simulink model "toa_wl00"  (Simulink 9.0)
settings: Solver=FixedStepDiscrete  StartTime=0.0  StopTime=inf  FixedStep=0.02  RelTol=1e-3  EnableMultiTasking=on
PreLoadFcn:
  | makefile_build_callback(bdroot,'toa_wl00.buildescription');
libraries: lib_CATutils_Utilities_ApplyName_v2 x3, package_instance x1, tip_assist_lib_support x1
settings Model: LogicAnalyzerSignalOrdering=5984164a-15a1-47b0-834b-00decfb9521f  MinMaxOverflowLogging=MinMaxAndOverflow  Creator=gulamhs  LastModifiedBy=CurriSD
settings DataIOCC: ExternalInput=[t,u]  SaveCompleteFinalSimState=on  SaveFormat=StructureWithTime  SaveOutput=off  SignalLogging=off  DSMLogging=off  SaveTime=off
settings OptimizationCC: DefaultParameterBehavior=Inlined  InlineInvariantSignals=on  EnhancedBackFolding=on  StrengthReduction=on  BitfieldContainerType=uchar_T  PassReuseOutputArgsAs=Individual arguments  ExpressionDepthLimit=2147483647  EfficientFloat2IntCast=on
settings DebuggingCC: SignalInfNanChecking=error  SignalRangeChecking=error  ReadBeforeWriteMsg=EnableAllAsError  WriteAfterWriteMsg=EnableAllAsError  WriteAfterReadMsg=EnableAllAsError  AlgebraicLoopMsg=error  ArtificialAlgebraicLoopMsg=error  SaveWithDisabledLinksMsg=error  SaveWithParameterizedLinksMsg=error  UnderspecifiedInitializationDetection=Simplified  MergeDetectMultiDrivingBlocksExec=error  BlockPriorityViolationMsg=error  SolverPrmCheckMsg=error  InheritedTsInSrcMsg=none  TasksWithSamePriorityMsg=error  SigSpecEnsureSampleTimeMsg=error  CheckMatrixSingularityMsg=error  IntegerOverflowMsg=error  ParameterUnderflowMsg=error  ParameterPrecisionLossMsg=none  FixptConstUnderflowMsg=error  FixptConstOverflowMsg=error  UnderSpecifiedDataTypeMsg=error  VectorMatrixConversionMsg=error  FcnCallInpInsideContextMsg=warning  UnconnectedInputMsg=error  UnconnectedOutputMsg=error  UnconnectedLineMsg=error  SFcnCompatibilityMsg=error  FrameProcessingCompatibilityMsg=warning  UniqueDataStoreMsg=error  BusObjectLabelMismatch=error  RootOutportRequireBusObject=error  AssertControl=DisableAll  ModelReferenceIOMsg=error  ModelReferenceVersionMismatchMessage=warning  ModelReferenceIOMismatchMessage=error  UnknownTsInhSupMsg=error  ModelReferenceDataLoggingMessage=error  StateNameClashWarn=warning  SimStateInterfaceChecksumMismatchMsg=error  StrictBusMsg=ErrorOnBusTreatedAsVector  BusNameAdapt=ErrorWithoutRepair  NonBusSignalsTreatedAsBus=error  SFInvalidInputDataAccessInChartInitDiag=error  SFNoUnconditionalDefaultTransitionDiag=error  SFTransitionOutsideNaturalParentDiag=error  SFUnreachableExecutionPathDiag=error  SFUndirectedBroadcastEventsDiag=error  SFExecutionAtInitializationDiag=warning  IntegerSaturationMsg=error
settings HardwareCC: ProdBitPerLong=64  ProdBitPerPointer=64  ProdBitPerSizeT=64  ProdBitPerPtrDiffT=64  ProdLargestAtomicInteger=Integer  ProdLargestAtomicFloat=Float  ProdIntDivRoundTo=Zero  ProdEndianess=LittleEndian  ProdWordSize=64  ProdHWDeviceType=Intel->x86-64 (Linux 64)
settings ModelReferenceCC: ParallelModelReferenceMATLABWorkerInit=Load Top Model  PropagateSignalLabelsOutOfModel=on
settings SFSimCC: SFSimEcho=off  SimGenImportedTypeDefs=on  MATLABDynamicMemAlloc=off
settings RTWCC: SystemTargetFile=cat_PkgArch.tlc  GenCodeOnly=on  GenerateMakefile=off  TemplateMakefile=cat_PkgArch_default_tmf  Description=R7a CAT Package Architecture Code Generation.  GenerateReport=on  RTWUseSimCustomCode=on  CodeProfilingSaveOptions=AllData  GenerateTraceReport=on  GenerateTraceReportSl=on  GenerateTraceReportSf=on  GenerateTraceReportEml=on  GenerateWebview=on  GenerateCodeMetricsReport=on  GenerateCodeReplacementReport=on
settings CodeAppCC: ForceParamTrailComments=on  IgnoreCustomStorageClasses=off  MaxIdLength=63  OperatorAnnotations=on  SimulinkDataObjDesc=on  SFDataObjDesc=on  MATLABFcnDesc=on  MangleLength=4  CustomSymbolStrType=$N$R$M  InsertBlockDesc=on  MATLABSourceComments=on  InternalIdentifier=Classic  ReqsInCode=on  UseSimReservedNames=on
settings STFCustomTargetCC: UtilityFuncGeneration=Shared location  MultiwordTypeDef=User defined  IncludeMdlTerminateFcn=off  CombineOutputUpdateFcns=on  SuppressErrorStatus=on  ERTCustomFileBanners=on  SupportAbsoluteTime=off  MultiInstanceERTCode=on  CodeInterfacePackaging=Reusable function  SupportComplex=off  SupportContinuousTime=off  SupportNonInlinedSFcns=off  RemoveResetFunc=on  SupportVariableSizeSignals=on  ParenthesesLevel=Maximum  MATLABClassNameForMDSCustomization=Simulink.SoftwareTarget.ERTCustomization  GRTInterface=off  GenerateSharedConstants=off  SystemTargetFile=cat_PkgArch.tlc
settings ERTTargetCC: UtilityFuncGeneration=Shared location  MultiwordTypeDef=User defined  MultiwordLength=2048  ParMdlRefBuildCompliant=off  CompOptLevelCompliant=off  ConcurrentExecutionCompliant=off  IncludeMdlTerminateFcn=off  SuppressErrorStatus=on  SupportAbsoluteTime=off  MultiInstanceERTCode=on  CodeInterfacePackaging=Reusable function  SupportComplex=off  SupportVariableSizeSignals=on  ParenthesesLevel=Maximum  ModelStepFunctionPrototypeControlCompliant=off  CPPClassGenCompliant=off  UseToolchainInfoCompliant=off  GenerateSharedConstants=off  MultiInstanceErrorCode=None  ERTSrcFileBannerTemplate=cat_code_template.cgt  ERTHdrFileBannerTemplate=cat_code_template.cgt  ERTDataSrcFileTemplate=cat_code_template.cgt  ERTDataHdrFileTemplate=cat_code_template.cgt  ERTCustomFileTemplate=cat_PkgArch_CFP.tlc  SuppressUnreachableDefaultCases=off  EnableUserReplacementTypes=on
settings MATStruct: int32=int32_t  int16=int16_t  int8=int8_t  uint32=uint32_t  uint16=uint16_t  uint8=uint8_t
settings CustomProperty: Value=Development
settings EnumStrPairs: String=Development
settings ConfigComp: CovMetricSettings=dwe  CovHtmlReporting=off  CovSaveCumulativeToWorkspaceVar=off  CovSaveSingleToWorkspaceVar=off  CovExternalEMLEnable=on

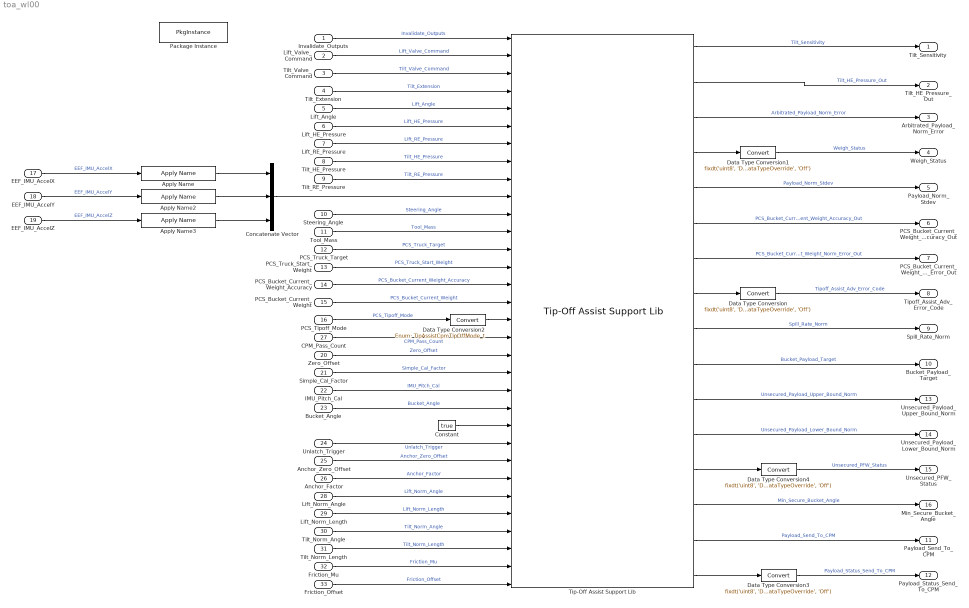
== system toa_wl00 ==
  Invalidate_Outputs : Inport
  Lift_Valve_Command : Inport  Port=2
  Tilt_Valve_Command : Inport  Port=3
  Tilt_Extension : Inport  Port=4
  Lift_Angle : Inport  Port=5
  Lift_HE_Pressure : Inport  Port=6
  Lift_RE_Pressure : Inport  Port=7
  Tilt_HE_Pressure : Inport  Port=8
  Tilt_RE_Pressure : Inport  Port=9
  Steering_Angle : Inport  Port=10
  Tool_Mass : Inport  Port=11
  PCS_Truck_Target : Inport  Port=12
  PCS_Truck_Start_Weight : Inport  Port=13
  PCS_Bucket_Current_Weight_Accuracy : Inport  Port=14
  PCS_Bucket_Current_Weight : Inport  Port=15
  PCS_Tipoff_Mode : Inport  Port=16
  EEF_IMU_AccelX : Inport  Port=17
  EEF_IMU_AccelY : Inport  Port=18
  EEF_IMU_AccelZ : Inport  Port=19
  Zero_Offset : Inport  Port=20
  Simple_Cal_Factor : Inport  Port=21
  IMU_Pitch_Cal : Inport  Port=22
  Bucket_Angle : Inport  Port=23
  Unlatch_Trigger : Inport  Port=24
  Anchor_Zero_Offset : Inport  Port=25
  Anchor_Factor : Inport  Port=26
  CPM_Pass_Count : Inport  Port=27
  Lift_Norm_Angle : Inport  Port=28
  Lift_Norm_Length : Inport  Port=29
  Tilt_Norm_Angle : Inport  Port=30
  Tilt_Norm_Length : Inport  Port=31
  Friction_Mu : Inport  Port=32
  Friction_Offset : Inport  Port=33
  Apply Name : lib_CATutils_Utilities_ApplyName_v2/Apply Name  sigLabel='toa_inImuAcclX'  enTst=true
  Apply Name2 : lib_CATutils_Utilities_ApplyName_v2/Apply Name  sigLabel='toa_inImuAcclY'  enTst=true
  Apply Name3 : lib_CATutils_Utilities_ApplyName_v2/Apply Name  sigLabel='toa_inImuAcclZ'  enTst=true
  Concatenate Vector : Concatenate  NumInputs=3  Mode=Multidimensional array
  Constant : Constant  Value=true  OutDataTypeStr=boolean  SampleTime=-1
  Data Type Conversion : DataTypeConversion  OutMin=[0]  OutMax=[6]  OutDataTypeStr=fixdt('uint8', 'DataTypeOverride', 'Off')
  Data Type Conversion1 : DataTypeConversion  OutMin=[0]  OutMax=[5]  OutDataTypeStr=fixdt('uint8', 'DataTypeOverride', 'Off')
  Data Type Conversion2 : DataTypeConversion  OutDataTypeStr=Enum: TipAssistCpmTipOffMode_t
  Data Type Conversion3 : DataTypeConversion  OutMin=[0]  OutMax=[5]  OutDataTypeStr=fixdt('uint8', 'DataTypeOverride', 'Off')
  Data Type Conversion4 : DataTypeConversion  OutMin=[0]  OutMax=[5]  OutDataTypeStr=fixdt('uint8', 'DataTypeOverride', 'Off')
  Package Instance : package_instance/PkgInstance  pkgName=toa_wl00  InitTaskTag=SSS_TID_INIT  tidHeader=sss_oel_defs.h  availModelRates={ '0.02', 'SSS_TID_20MSEC' }  Platform=Any (No Hardware Dependencies)  TPUA_TCR1=12800  TPUA_TCR2=200  TPUB_TCR1=12800  TPUB_TCR2=200
  Tip-Off Assist Support Lib : tip_assist_lib_support/Tip-Off Assist Support Lib
  Tilt_Sensitivity : Outport
  Tilt_HE_Pressure_Out : Outport  Port=2
  Arbitrated_Payload_Norm_Error : Outport  Port=3
  Weigh_Status : Outport  Port=4
  Payload_Norm_Stdev : Outport  Port=5
  PCS_Bucket_Current_Weight_Accuracy_Out : Outport  Port=6
  PCS_Bucket_Current_Weight_Norm_Error_Out : Outport  Port=7
  Tipoff_Assist_Adv_Error_Code : Outport  Port=8
  Spill_Rate_Norm : Outport  Port=9
  Bucket_Payload_Target : Outport  Port=10
  Payload_Send_To_CPM : Outport  Port=11
  Payload_Status_Send_To_CPM : Outport  Port=12
  Unsecured_Payload_Upper_Bound_Norm : Outport  Port=13
  Unsecured_Payload_Lower_Bound_Norm : Outport  Port=14
  Unsecured_PFW_Status : Outport  Port=15
  Min_Secure_Bucket_Angle : Outport  Port=16
  wires:
  Steering_Angle/1 -> Tip-Off Assist Support Lib/11  "Steering_Angle"
  Tool_Mass/1 -> Tip-Off Assist Support Lib/12  "Tool_Mass"
  PCS_Truck_Target/1 -> Tip-Off Assist Support Lib/13  "PCS_Truck_Target"
  PCS_Truck_Start_Weight/1 -> Tip-Off Assist Support Lib/14  "PCS_Truck_Start_Weight"
  PCS_Bucket_Current_Weight_Accuracy/1 -> Tip-Off Assist Support Lib/15  "PCS_Bucket_Current_Weight_Accuracy"
  PCS_Bucket_Current_Weight/1 -> Tip-Off Assist Support Lib/16  "PCS_Bucket_Current_Weight"
  Tip-Off Assist Support Lib/1 -> Tilt_Sensitivity/1  "Tilt_Sensitivity"
  Tip-Off Assist Support Lib/2 -> Tilt_HE_Pressure_Out/1  "Tilt_HE_Pressure_Out"
  Tip-Off Assist Support Lib/3 -> Arbitrated_Payload_Norm_Error/1  "Arbitrated_Payload_Norm_Error"
  Tip-Off Assist Support Lib/5 -> Payload_Norm_Stdev/1  "Payload_Norm_Stdev"
  Tip-Off Assist Support Lib/6 -> PCS_Bucket_Current_Weight_Accuracy_Out/1  "PCS_Bucket_Current_Weight_Accuracy_Out"
  Tip-Off Assist Support Lib/7 -> PCS_Bucket_Current_Weight_Norm_Error_Out/1  "PCS_Bucket_Current_Weight_Norm_Error_Out"
  Tip-Off Assist Support Lib/9 -> Spill_Rate_Norm/1  "Spill_Rate_Norm"
  Apply Name2/1 -> Concatenate Vector/2
  Apply Name/1 -> Concatenate Vector/1
  Apply Name3/1 -> Concatenate Vector/3
  EEF_IMU_AccelX/1 -> Apply Name/1  "EEF_IMU_AccelX"
  EEF_IMU_AccelY/1 -> Apply Name2/1  "EEF_IMU_AccelY"
  EEF_IMU_AccelZ/1 -> Apply Name3/1  "EEF_IMU_AccelZ"
  Concatenate Vector/1 -> Tip-Off Assist Support Lib/10
  PCS_Tipoff_Mode/1 -> Data Type Conversion2/1  "PCS_Tipoff_Mode"
  Tip-Off Assist Support Lib/8 -> Data Type Conversion/1
  Data Type Conversion/1 -> Tipoff_Assist_Adv_Error_Code/1  "Tipoff_Assist_Adv_Error_Code"
  Tip-Off Assist Support Lib/4 -> Data Type Conversion1/1
  Data Type Conversion1/1 -> Weigh_Status/1  "Weigh_Status"
  Data Type Conversion2/1 -> Tip-Off Assist Support Lib/17
  Data Type Conversion3/1 -> Payload_Status_Send_To_CPM/1  "Payload_Status_Send_To_CPM"
  Invalidate_Outputs/1 -> Tip-Off Assist Support Lib/1  "Invalidate_Outputs"
  Lift_Valve_Command/1 -> Tip-Off Assist Support Lib/2  "Lift_Valve_Command"
  Tilt_Valve_Command/1 -> Tip-Off Assist Support Lib/3  "Tilt_Valve_Command"
  Tilt_Extension/1 -> Tip-Off Assist Support Lib/4  "Tilt_Extension"
  Lift_Angle/1 -> Tip-Off Assist Support Lib/5  "Lift_Angle"
  Lift_HE_Pressure/1 -> Tip-Off Assist Support Lib/6  "Lift_HE_Pressure"
  Lift_RE_Pressure/1 -> Tip-Off Assist Support Lib/7  "Lift_RE_Pressure"
  Tilt_HE_Pressure/1 -> Tip-Off Assist Support Lib/8  "Tilt_HE_Pressure"
  Tilt_RE_Pressure/1 -> Tip-Off Assist Support Lib/9  "Tilt_RE_Pressure"
  Zero_Offset/1 -> Tip-Off Assist Support Lib/19  "Zero_Offset"
  Simple_Cal_Factor/1 -> Tip-Off Assist Support Lib/20  "Simple_Cal_Factor"
  IMU_Pitch_Cal/1 -> Tip-Off Assist Support Lib/21  "IMU_Pitch_Cal"
  Bucket_Angle/1 -> Tip-Off Assist Support Lib/22  "Bucket_Angle"
  Unlatch_Trigger/1 -> Tip-Off Assist Support Lib/24  "Unlatch_Trigger"
  Constant/1 -> Tip-Off Assist Support Lib/23
  Anchor_Zero_Offset/1 -> Tip-Off Assist Support Lib/25  "Anchor_Zero_Offset"
  Anchor_Factor/1 -> Tip-Off Assist Support Lib/26  "Anchor_Factor"
  Tip-Off Assist Support Lib/10 -> Bucket_Payload_Target/1  "Bucket_Payload_Target"
  CPM_Pass_Count/1 -> Tip-Off Assist Support Lib/18  "CPM_Pass_Count"
  Lift_Norm_Angle/1 -> Tip-Off Assist Support Lib/27  "Lift_Norm_Angle"
  Lift_Norm_Length/1 -> Tip-Off Assist Support Lib/28  "Lift_Norm_Length"
  Tilt_Norm_Angle/1 -> Tip-Off Assist Support Lib/29  "Tilt_Norm_Angle"
  Tilt_Norm_Length/1 -> Tip-Off Assist Support Lib/30  "Tilt_Norm_Length"
  Data Type Conversion4/1 -> Unsecured_PFW_Status/1  "Unsecured_PFW_Status"
  Tip-Off Assist Support Lib/16 -> Data Type Conversion3/1
  Tip-Off Assist Support Lib/11 -> Unsecured_Payload_Upper_Bound_Norm/1  "Unsecured_Payload_Upper_Bound_Norm"
  Tip-Off Assist Support Lib/12 -> Unsecured_Payload_Lower_Bound_Norm/1  "Unsecured_Payload_Lower_Bound_Norm"
  Tip-Off Assist Support Lib/13 -> Data Type Conversion4/1
  Tip-Off Assist Support Lib/14 -> Min_Secure_Bucket_Angle/1  "Min_Secure_Bucket_Angle"
  Tip-Off Assist Support Lib/15 -> Payload_Send_To_CPM/1  "Payload_Send_To_CPM"
  Friction_Mu/1 -> Tip-Off Assist Support Lib/31  "Friction_Mu"
  Friction_Offset/1 -> Tip-Off Assist Support Lib/32  "Friction_Offset"
